simulink model "rlc_power_measurement"  (R2025b)
settings: Solver=ode1  StartTime=0.0  StopTime=0.1  FixedStep=1/50000  RelTol=1e-3
libraries: spsRMSLib x3, spsPowerLib x2, spsSeriesRLCBranchLib x2, spsVoltageMeasurementLib x2, spsACVoltageSourceLib x1, spsCurrentMeasurementLib x1, sps_lib x1
settings Model: Creator=Supervisor  LastModifiedBy=Supervisor

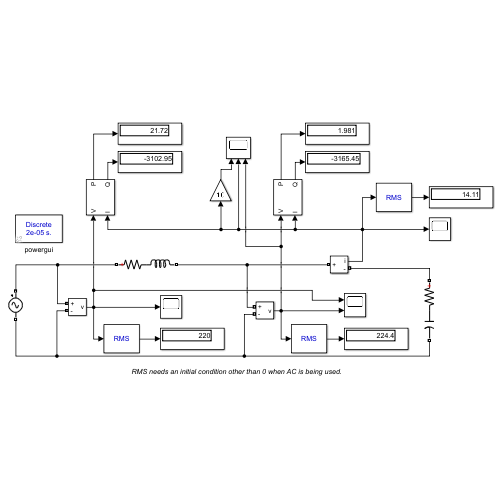
[thumbnail: Simulink's stored preview of the top-level diagram]
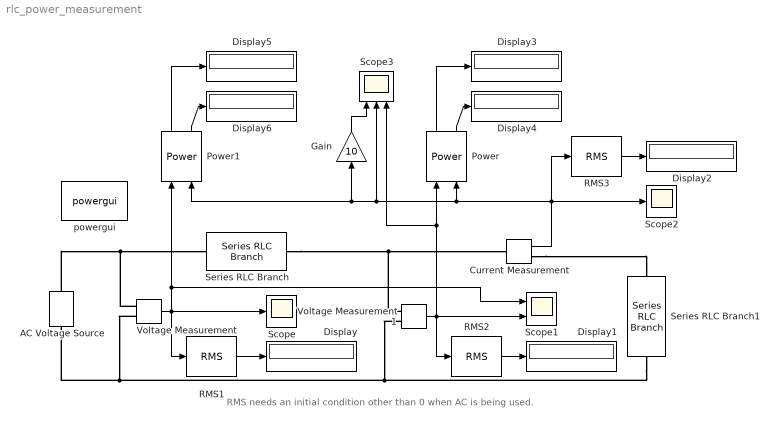
== system rlc_power_measurement ==
  note: RMS needs an initial condition other than 0 when AC is being used.
  AC Voltage Source : spsACVoltageSourceLib/AC Voltage Source  Amplitude=sqrt(2)*220  Phase=0  Frequency=50  SampleTime=0  Measurements=None  BusType=swing  Pref=10e3  Qref=0  Qmin=-inf  Qmax=+inf
  Current Measurement : spsCurrentMeasurementLib/Current Measurement  PhasorSimulation=off  OutputType=Complex  PSBequivalent=0
  Display{,1..6} (7 alike) : Display
      Display4 settings: Format=bank
      Display6 settings: Format=bank
  Gain : Gain  Gain=10
  Power : spsPowerLib/Power  Freq=50  Vinit=[1, 0]  Iinit=[1, 0]  Ts=0
  Power1 : spsPowerLib/Power  Freq=50  Vinit=[1, 0]  Iinit=[1, 0]  Ts=0
  RMS1 : spsRMSLib/RMS  TrueRMS=on  Freq=50  RMSInit=120  Ts=0
  RMS2 : spsRMSLib/RMS  TrueRMS=on  Freq=50  RMSInit=120  Ts=0
  RMS3 : spsRMSLib/RMS  TrueRMS=on  Freq=50  RMSInit=1  Ts=0
  Scope : Scope
      settings: ActiveDisplayYMinimum=-1  ActiveDisplayYMaximum=1
  Scope1 : Scope  NumInputPorts=2
      settings: ActiveDisplayYMinimum=-388.9087296526011  ActiveDisplayYMaximum=388.9087296526011
  Scope2 : Scope
      settings: ActiveDisplayYMinimum=-1  ActiveDisplayYMaximum=1  DataLoggingVariableName=ScopeData2
  Scope3 : Scope  NumInputPorts=3
      settings: ActiveDisplayYMinimum=-424.20353599939045  ActiveDisplayYMaximum=453.60896927018047  DataLoggingVariableName=ScopeData3
  Series RLC Branch : spsSeriesRLCBranchLib/Series RLC Branch  LConnTagsString=__new0  RConnTagsString=__new0  BranchType=RL  Resistance=0.1  Inductance=1e-3  SetiL0=off  InitialCurrent=0  Capacitance=10e-6  Setx0=off  InitialVoltage=0  Measurements=None
  Series RLC Branch1 : spsSeriesRLCBranchLib/Series RLC Branch  LConnTagsString=__new0  RConnTagsString=__new0  BranchType=RC  Resistance=0.01  Inductance=1e-3  SetiL0=off  InitialCurrent=0  Capacitance=200e-6  Setx0=off  InitialVoltage=0  Measurements=None
  Voltage Measurement : spsVoltageMeasurementLib/Voltage Measurement  PhasorSimulation=off  OutputType=Complex  PSBequivalent=0
  Voltage Measurement1 : spsVoltageMeasurementLib/Voltage Measurement  PhasorSimulation=off  OutputType=Complex  PSBequivalent=0
  powergui : sps_lib/powergui  Priority=1  SimulationMode=Discrete  SampleTime=1/50000  frequency=60  Iterations=50  frequencyindice=50  Pbase=100e6  ErrMax=1e-4  UnitsV=kV  UnitsW=MW  buscounter=0  FunctionMessages=off  echomessages=off  EnableUseOfTLC=off  CurrentSourceSwitches=off  DisableSnubberDevices=off  DisableRonSwitches=off  DisableVfSwitches=off  DisplayEquations=off  AutomaticDiscreteSolvers=off  SolverType=Tustin/Backward Euler (TBE)  Interpol=off  ExternalGateDelay=off  methode=off  Ts=10  x0status=zero  SPID=off  SwTol=0  HookPort=off  NonlinearTolerance=1e-4  nMaxIteration=100  ContinueOnMaxIteration=off  RestoreLinks=warning  ResistiveCurrentMeasurement=off  Frange=[0:2:500]  Ylog=off  Xlog=on  ShowGrid=off  save=off  variable=ZData  structure=0  ZoomFFT=off  StartTime=0.0  cycles=1  DisplayStyle=1  fundamental=60  FreqAxis=off  MaxFrequency=1000  frequencyindicesteady=1  RmsSteady=1  display=off
  wires:
  Voltage Measurement/1 -> RMS1/1, Scope1/1, Power1/1, Scope/1
  Voltage Measurement1/1 -> Scope1/2, Scope3/3, Power/1, RMS2/1
  Current Measurement/1 -> Power1/2, Gain/1, Scope3/2, Power/2, RMS3/1, Scope2/1
  RMS1/1 -> Display/1
  RMS2/1 -> Display1/1
  RMS3/1 -> Display2/1
  Power/1 -> Display3/1
  Power/2 -> Display4/1
  Power1/2 -> Display6/1
  Power1/1 -> Display5/1
  Gain/1 -> Scope3/1
  connections:
  AC Voltage Source/RConn1 -- Voltage Measurement/LConn1 -- Series RLC Branch/LConn1
  Series RLC Branch/RConn1 -- Voltage Measurement1/LConn1 -- Current Measurement/LConn1
  Current Measurement/RConn1 -- Series RLC Branch1/LConn1
  Series RLC Branch1/RConn1 -- Voltage Measurement1/LConn2 -- Voltage Measurement/LConn2 -- AC Voltage Source/LConn1
